simulink model "fsm_simulink"  (R2026b)
settings: Solver=VariableStepAuto  StopTime=20
libraries: fuzblock x2
settings Model: Creator=Hp  LastModifiedBy=Mohammad

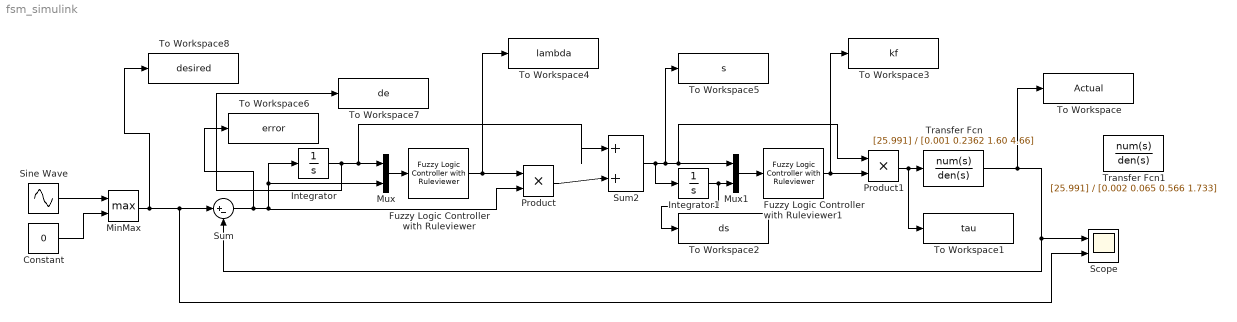
== system fsm_simulink ==
  Constant : Constant  Value=0  SampleTime=-1
  Fuzzy Logic Controller with Ruleviewer : fuzblock/Fuzzy Logic  Controller  with Ruleviewer  FIS=slide  Ts=2
  Fuzzy Logic Controller with Ruleviewer1 : fuzblock/Fuzzy Logic  Controller  with Ruleviewer  FIS=slide  Ts=2
  Integrator : Integrator
  Integrator1 : Integrator
  MinMax : MinMax  Function=max  Inputs=2
  Mux : Mux  Inputs=2
  Mux1 : Mux  Inputs=2
  Product : Product
  Product1 : Product
  Scope : Scope  NumInputPorts=2
      settings: ActiveDisplayYMinimum=-2.76976  ActiveDisplayYMaximum=22.52968
  Sine Wave : Sin  Amplitude=20  Phase=3.14
  Sum : Sum  Inputs=|+-
  Sum2 : Sum  Inputs=|++
  To Workspace : ToWorkspace  VariableName=Actual  SaveFormat=Timeseries  SampleTime=-1
  To Workspace1 : ToWorkspace  VariableName=tau  SaveFormat=Timeseries  SampleTime=-1
  To Workspace2 : ToWorkspace  VariableName=ds  SaveFormat=Timeseries  SampleTime=-1
  To Workspace3 : ToWorkspace  VariableName=kf  SaveFormat=Timeseries  SampleTime=-1
  To Workspace4 : ToWorkspace  VariableName=lambda  SaveFormat=Timeseries  SampleTime=-1
  To Workspace5 : ToWorkspace  VariableName=s  SaveFormat=Timeseries  SampleTime=-1
  To Workspace6 : ToWorkspace  VariableName=error  SaveFormat=Timeseries  SampleTime=-1
  To Workspace7 : ToWorkspace  VariableName=de  SaveFormat=Timeseries  SampleTime=-1
  To Workspace8 : ToWorkspace  VariableName=desired  SaveFormat=Timeseries  SampleTime=-1
  Transfer Fcn : TransferFcn  Numerator=[25.991]  Denominator=[0.001 0.2362 1.60 4.66]
  Transfer Fcn1 : TransferFcn  Numerator=[25.991]  Denominator=[0.002 0.065 0.566 1.733]
  wires:
  Fuzzy Logic Controller with Ruleviewer1/1 -> Product1/2, To Workspace3/1
  Product1/1 -> Transfer Fcn/1, To Workspace1/1
  Integrator1/1 -> To Workspace2/1, Mux1/2
  Sum2/1 -> Integrator1/1, To Workspace5/1, Product1/1, Mux1/1
  Integrator/1 -> To Workspace7/1, Sum2/1, Mux/1
  Mux/1 -> Fuzzy Logic Controller with Ruleviewer/1
  Mux1/1 -> Fuzzy Logic Controller with Ruleviewer1/1
  Sum/1 -> To Workspace6/1, Product/2, Mux/2, Integrator/1
  Product/1 -> Sum2/2
  Sine Wave/1 -> MinMax/1
  MinMax/1 -> To Workspace8/1, Scope/2, Sum/1
  Transfer Fcn/1 -> To Workspace/1, Scope/1, Sum/2
  Fuzzy Logic Controller with Ruleviewer/1 -> To Workspace4/1, Product/1
  Constant/1 -> MinMax/2
